simulink model "scalar_ramp_noise"  (Simulink 4.00)
settings: Solver=ode45  SolverMode=SingleTasking  StartTime=0.0  StopTime=10.0  FixedStep=1  RelTol=1e-3
undefined symbols (not defined in the file or in its folder): recursive_avg
libraries: simulink3 x1
settings Model: OptimizeBlockIOStorage=off  BlockReductionOpt=off

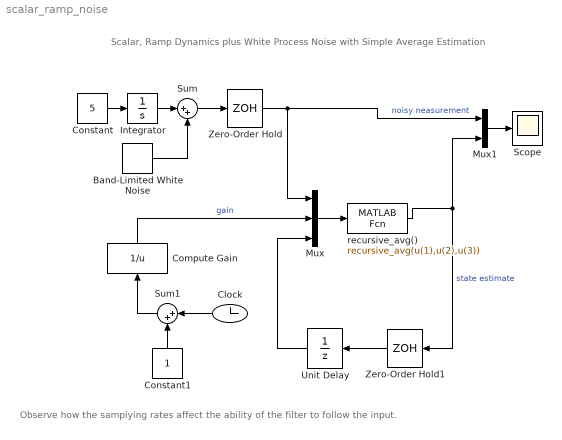
== system scalar_ramp_noise ==
  note: Scalar, Ramp Dynamics
      | plus White Process Noise
      | with Simple Average Estimation
  note: Observe how the samplying rates affect the ability of
      | the filter to follow the input.
  Band-Limited White Noise : simulink3/Sources/Band-Limited White Noise  Cov=[0.1]  Ts=1  seed=[23341+floor(1000*rand(1))]
  Clock : Clock
  Compute Gain : MATLABFcn  Orientation=up  MATLABFcn=1/u  OutputDimensions=-1  OutputSignalType=auto  Output1D=off
  Constant : Constant  Value=5
  Constant1 : Constant  Orientation=up  Value=1
  Integrator : Integrator  ExternalReset=none  InitialConditionSource=internal  InitialCondition=0  LimitOutput=off  UpperSaturationLimit=inf  LowerSaturationLimit=-inf  ShowSaturationPort=off  ShowStatePort=off  AbsoluteTolerance=auto
  Mux : Mux  Inputs=3
  Mux1 : Mux  Inputs=2
  Scope : Scope
      settings: TimeRange=auto  YMin=-2.5  YMax=32.5  SaveToWorkspace=off  SaveName=ScopeData  LimitDataPoints=on  MaxDataPoints=5000
  Sum : Sum  Inputs=|++  SaturateOnIntegerOverflow=on
  Sum1 : Sum  Orientation=left  Inputs=|++  SaturateOnIntegerOverflow=on
  Unit Delay : UnitDelay  Orientation=left  X0=0  SampleTime=-1
  Zero-Order Hold : ZeroOrderHold  SampleTime=.1
  Zero-Order Hold1 : ZeroOrderHold  Orientation=left  SampleTime=1
  recursive_avg() : MATLABFcn  MATLABFcn=recursive_avg(u(1),u(2),u(3))  OutputDimensions=-1  OutputSignalType=auto  Output1D=on
  wires:
  Band-Limited White Noise/1 -> Sum/2
  Constant/1 -> Integrator/1
  Sum/1 -> Zero-Order Hold/1
  recursive_avg()/1 -> Mux1/2, Zero-Order Hold1/1  "state estimate"
  Mux/1 -> recursive_avg()/1
  Clock/1 -> Sum1/1
  Constant1/1 -> Sum1/2
  Sum1/1 -> Compute Gain/1
  Zero-Order Hold/1 -> Mux/1, Mux1/1  "noisy neasurement"
  Zero-Order Hold1/1 -> Unit Delay/1
  Compute Gain/1 -> Mux/2  "gain"
  Unit Delay/1 -> Mux/3
  Integrator/1 -> Sum/1
  Mux1/1 -> Scope/1
